simulink model "ACC_FFNN_trainbfg_30_30_30_Nor_Sat_Jan_24_RepFast"  (R2021a)
settings: Solver=FixedStepAuto  StartTime=0.0  StopTime=T  RelTol=1e-3
InitFcn:
  | seed = randi(10000);
StartFcn:
  | seed = randi(10000);
undefined symbols (not defined in the file): amax_ego, amin_ego, patch_sig, safe_patch_sig, sw, t_gap, Ts, v0_ego, v0_lead, v_set, x0_ego, x0_lead, x_gain, x_offset, y_gain, y_offset
libraries: neural x95, simulink x3
(part 1 of 5)
settings Model: Creator=The MathWorks, Inc.  LastModifiedBy=deyun
settings SolverCC: AlgebraicLoopSolver=TrustRegion
settings DataIOCC: ReturnWorkspaceOutputs=off
settings DebuggingCC: ArithmeticOperatorsInVariantConditions=warning
settings SFSimCC: SimUseLocalCustomCode=off  CustomCodeUndefinedFunction=UseInterfaceOnly
settings RTWCC: RTWUseLocalCustomCode=off
settings CodeAppCC: StateflowObjectComments=on
settings ConfigComp: CovBoundaryAbsTol=1.0e-5

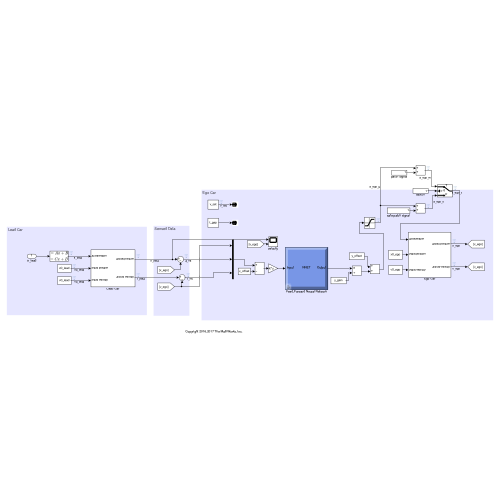
[thumbnail: Simulink's stored preview of the top-level diagram]
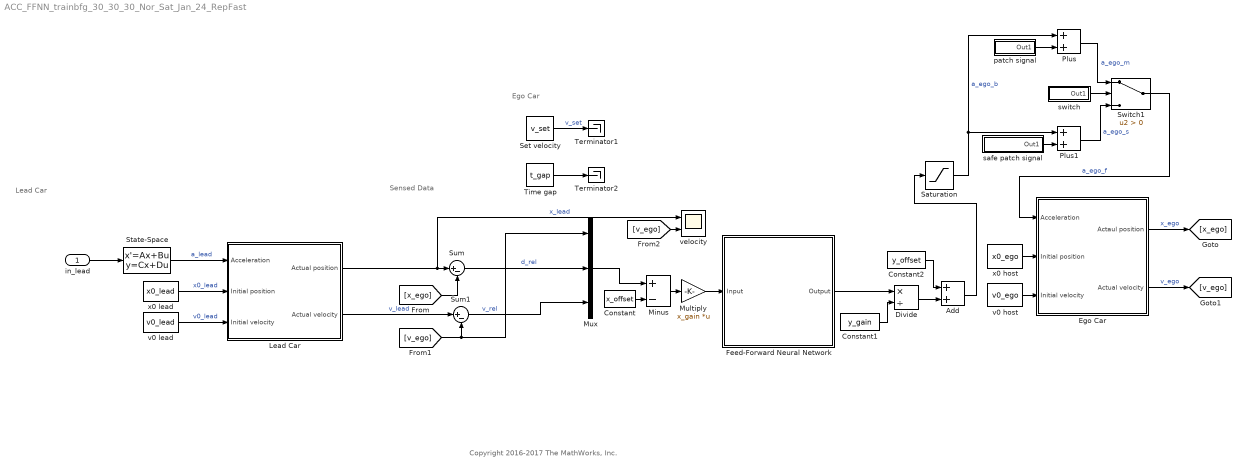
== system ACC_FFNN_trainbfg_30_30_30_Nor_Sat_Jan_24_RepFast ==
  note: Sensed Data
  note: Lead Car
  note: Ego Car
  note: Copyright 2016-2017 The MathWorks, Inc.
  in_lead : Inport
  Add : Sum
  Constant : Constant  Value=x_offset
  Constant1 : Constant  Value=y_gain
  Constant2 : Constant  Value=y_offset
  Divide : Product  Inputs=*/
  Ego Car : Subsystem
  Feed-Forward Neural Network : Subsystem
      mask help: Feed-Forward Neural Network
      mask Display: e = 0.06;c1 = [120 150 230]/255;c2 = ([120 150 230]+0)/383;c3 = ([120 150 230]+128)/383;patch([0 1 1 0],[0 0 1 1],c1);patch([0 1 1 1-e 1-e 0+e],[0 0 1 1-e 0+e 0+e],c2);patch([0 0 1 1-e 0+e 0+e],[0 1 1 1-e 1-e 0+e],c3);plot([0 1 1 0 0],[0 0 1 1 0]);fprintf('NNET');port_label('input',1,' Input');port_label('output',1,'Output ');
  Lead Car : Subsystem
  Minus : Sum  Inputs=+-
  Multiply : Gain  Gain=x_gain  Multiplication=Matrix(K*u)
  Mux : Mux  Inputs=3
  Plus : Sum
  Plus1 : Sum
  Saturation : Saturate  UpperLimit=amax_ego  LowerLimit=amin_ego
  Set velocity : Constant  Value=v_set  SampleTime=Ts
  State-Space : StateSpace  A=-10  B=10  D=0  InitialCondition=0
  Sum : Sum  Inputs=|+-
  Sum1 : Sum  Inputs=|+-
  Switch1 : Switch  Criteria=u2 > Threshold
  Terminator1 : Terminator
  Terminator2 : Terminator
  Time gap : Constant  Value=t_gap  SampleTime=Ts
  patch signal : Subsystem
  safe patch signal : Subsystem
  switch : Subsystem
  v0 host : Constant  Value=v0_ego  SampleTime=Ts
  v0 lead : Constant  Value=v0_lead  SampleTime=Ts
  velocity : Scope  NumInputPorts=2
  x0 host : Constant  Value=x0_ego  SampleTime=Ts
  x0 lead : Constant  Value=x0_lead  SampleTime=Ts
  wires:
  x0 lead/1 -> Lead Car/2(Initial position)  "x0_lead"
  v0 lead/1 -> Lead Car/3(Initial velocity)  "v0_lead"
  x0 host/1 -> Ego Car/2(Initial position)
  v0 host/1 -> Ego Car/3(Initial velocity)
  Feed-Forward Neural Network/1(Output) -> Divide/1
  Lead Car/1(Actual position) -> velocity/1, Sum/1  "x_lead"
  Sum1/1 -> Mux/3  "v_rel"
  State-Space/1 -> Lead Car/1(Acceleration)  "a_lead"
  Lead Car/2(Actual velocity) -> Sum1/1  "v_lead"
  in_lead/1 -> State-Space/1
  Mux/1 -> Minus/1
  Add/1 -> Saturation/1
  Multiply/1 -> Feed-Forward Neural Network/1(Input)
  Set velocity/1 -> Terminator1/1  "v_set"
  Time gap/1 -> Terminator2/1
  Constant/1 -> Minus/2
  Minus/1 -> Multiply/1
  Constant1/1 -> Divide/2
  Divide/1 -> Add/2
  Constant2/1 -> Add/1
  Ego Car/1(Actaul position) -> [x_ego]  "x_ego"
  [x_ego] -> Sum/2
  Ego Car/2(Actual velocity) -> [v_ego]  "v_ego"
  [v_ego] -> Mux/1, Sum1/2
  [v_ego] -> velocity/2
  Sum/1 -> Mux/2  "d_rel"
  Plus/1 -> Switch1/1  "a_ego_m"
  Plus1/1 -> Switch1/3  "a_ego_s"
  Switch1/1 -> Ego Car/1(Acceleration)  "a_ego_f"
  Saturation/1 -> Plus/1, Plus1/1  "a_ego_b"
  patch signal/1(Out1) -> Plus/2
  safe patch signal/1(Out1) -> Plus1/2
  switch/1(Out1) -> Switch1/2

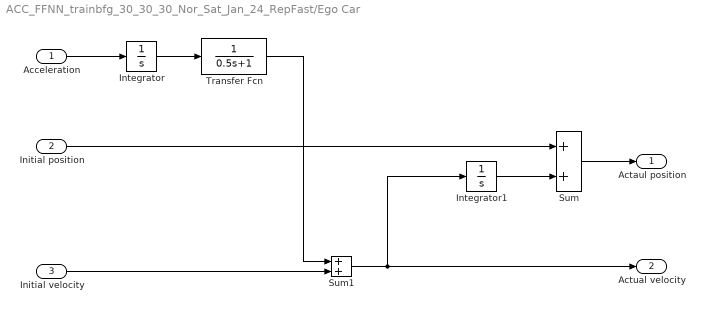
== system ACC_FFNN_trainbfg_30_30_30_Nor_Sat_Jan_24_RepFast/Ego Car ==
  Acceleration : Inport
  Initial position : Inport  Port=2
  Initial velocity : Inport  Port=3
  Integrator : Integrator
  Integrator1 : Integrator
  Sum : Sum
  Sum1 : Sum
  Transfer Fcn : TransferFcn  Denominator=[0.5 1]
  Actaul position : Outport  VectorParamsAs1DForOutWhenUnconnected=off
  Actual velocity : Outport  Port=2  VectorParamsAs1DForOutWhenUnconnected=off
  wires:
  Sum1/1 -> Integrator1/1, Actual velocity/1
  Initial velocity/1 -> Sum1/2
  Sum/1 -> Actaul position/1
  Transfer Fcn/1 -> Sum1/1
  Integrator/1 -> Transfer Fcn/1
  Acceleration/1 -> Integrator/1
  Initial position/1 -> Sum/1
  Integrator1/1 -> Sum/2

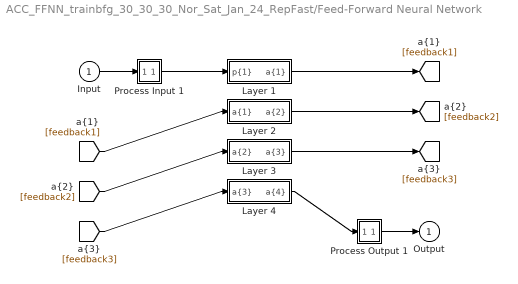
== system ACC_FFNN_trainbfg_30_30_30_Nor_Sat_Jan_24_RepFast/Feed-Forward Neural Network ==
  Input : Inport  PortDimensions=3
      mask Display: e = 0.06;c1 = [120 230 180]/255;c2 = ([120 230 180]+0)/(256+128);c3 = ([120 230 180]+128)/(256+128);patch([0 1 1 0],[0 0 1 1],c1);patch([0 1 1 1-e 1-e 0+e],[0 0 1 1-e 0+e 0+e],c2);patch([0 0 1 1-e 0+e 0+e],[0 1 1 1-e 1-e 0+e],c3);plot([0 1 1 0 0],[0 0 1 1 0]);
  Layer 1 : Subsystem
      mask Display: e = 0.06;c1 = [120 150 230]/255;c2 = ([120 150 230]+0)/383;c3 = ([120 150 230]+128)/383;patch([0 1 1 0],[0 0 1 1],c1);patch([0 1 1 1-e 1-e 0+e],[0 0 1 1-e 0+e 0+e],c2);patch([0 0 1 1-e 0+e 0+e],[0 1 1 1-e 1-e 0+e],c3);plot([0 1 1 0 0],[0 0 1 1 0]);
  Layer 2 : Subsystem
      mask Display: e = 0.06;c1 = [120 150 230]/255;c2 = ([120 150 230]+0)/383;c3 = ([120 150 230]+128)/383;patch([0 1 1 0],[0 0 1 1],c1);patch([0 1 1 1-e 1-e 0+e],[0 0 1 1-e 0+e 0+e],c2);patch([0 0 1 1-e 0+e 0+e],[0 1 1 1-e 1-e 0+e],c3);plot([0 1 1 0 0],[0 0 1 1 0]);
  Layer 3 : Subsystem
      mask Display: e = 0.06;c1 = [120 150 230]/255;c2 = ([120 150 230]+0)/383;c3 = ([120 150 230]+128)/383;patch([0 1 1 0],[0 0 1 1],c1);patch([0 1 1 1-e 1-e 0+e],[0 0 1 1-e 0+e 0+e],c2);patch([0 0 1 1-e 0+e 0+e],[0 1 1 1-e 1-e 0+e],c3);plot([0 1 1 0 0],[0 0 1 1 0]);
  Layer 4 : Subsystem
      mask Display: e = 0.06;c1 = [120 150 230]/255;c2 = ([120 150 230]+0)/383;c3 = ([120 150 230]+128)/383;patch([0 1 1 0],[0 0 1 1],c1);patch([0 1 1 1-e 1-e 0+e],[0 0 1 1-e 0+e 0+e],c2);patch([0 0 1 1-e 0+e 0+e],[0 1 1 1-e 1-e 0+e],c3);plot([0 1 1 0 0],[0 0 1 1 0]);
  Process Input 1 : Subsystem
      mask Display: e = 0.06;c1 = [120 150 230]/255;c2 = ([120 150 230]+0)/383;c3 = ([120 150 230]+128)/383;patch([0 1 1 0],[0 0 1 1],c1);patch([0 1 1 1-e 1-e 0+e],[0 0 1 1-e 0+e 0+e],c2);patch([0 0 1 1-e 0+e 0+e],[0 1 1 1-e 1-e 0+e],c3);plot([0 1 1 0 0],[0 0 1 1 0]);
  Process Output 1 : Subsystem
      mask Display: e = 0.06;c1 = [120 150 230]/255;c2 = ([120 150 230]+0)/383;c3 = ([120 150 230]+128)/383;patch([0 1 1 0],[0 0 1 1],c1);patch([0 1 1 1-e 1-e 0+e],[0 0 1 1-e 0+e 0+e],c2);patch([0 0 1 1-e 0+e 0+e],[0 1 1 1-e 1-e 0+e],c3);plot([0 1 1 0 0],[0 0 1 1 0]);
  Output : Outport  InitialOutput=0
      mask Display: e = 0.06;c1 = [120 230 180]/255;c2 = ([120 230 180]+0)/(256+128);c3 = ([120 230 180]+128)/(256+128);patch([0 1 1 0],[0 0 1 1],c1);patch([0 1 1 1-e 1-e 0+e],[0 0 1 1-e 0+e 0+e],c2);patch([0 0 1 1-e 0+e 0+e],[0 1 1 1-e 1-e 0+e],c3);plot([0 1 1 0 0],[0 0 1 1 0]);
  wires:
  Input/1 -> Process Input 1/1(x)
  Process Output 1/1(y) -> Output/1
  Process Input 1/1(p) -> Layer 1/1("p{1}")
  Layer 1/1("a{1}") -> [feedback1]
  [feedback1] -> Layer 2/1("a{1} ")
  Layer 2/1("a{2}") -> [feedback2]
  [feedback2] -> Layer 3/1("a{2} ")
  Layer 3/1("a{3}") -> [feedback3]
  [feedback3] -> Layer 4/1("a{3} ")
  Layer 4/1("a{4}") -> Process Output 1/1(a)

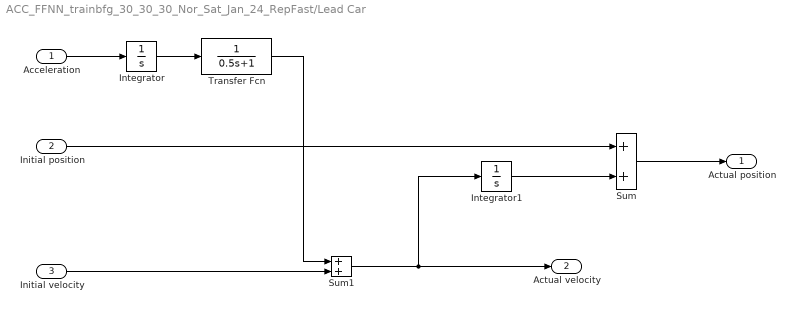
== system ACC_FFNN_trainbfg_30_30_30_Nor_Sat_Jan_24_RepFast/Lead Car ==
  Acceleration : Inport
  Initial position : Inport  Port=2
  Initial velocity : Inport  Port=3
  Integrator : Integrator
  Integrator1 : Integrator
  Sum : Sum
  Sum1 : Sum
  Transfer Fcn : TransferFcn  Denominator=[0.5 1]
  Actual position : Outport  VectorParamsAs1DForOutWhenUnconnected=off
  Actual velocity : Outport  Port=2  VectorParamsAs1DForOutWhenUnconnected=off
  wires:
  Transfer Fcn/1 -> Sum1/1
  Initial velocity/1 -> Sum1/2
  Sum/1 -> Actual position/1
  Integrator/1 -> Transfer Fcn/1
  Sum1/1 -> Integrator1/1, Actual velocity/1
  Acceleration/1 -> Integrator/1
  Initial position/1 -> Sum/1
  Integrator1/1 -> Sum/2

== system ACC_FFNN_trainbfg_30_30_30_Nor_Sat_Jan_24_RepFast/patch signal ==
  Sample index : simulink/Sources/Counter Limited  uplimit=numel(patch_sig)-1  tsamp=Ts
  Sample value : LookupNDDirect  NumberOfTableDimensions=1  Table=patch_sig  DiagnosticForOutOfRangeInput=None
  Out1 : Outport
  wires:
  Sample index/1 -> Sample value/1
  Sample value/1 -> Out1/1

== system ACC_FFNN_trainbfg_30_30_30_Nor_Sat_Jan_24_RepFast/safe patch signal ==
  Sample index : simulink/Sources/Counter Limited  uplimit=numel(safe_patch_sig)-1  tsamp=Ts
  Sample value : LookupNDDirect  NumberOfTableDimensions=1  Table=safe_patch_sig  DiagnosticForOutOfRangeInput=None
  Out1 : Outport
  wires:
  Sample index/1 -> Sample value/1
  Sample value/1 -> Out1/1

== system ACC_FFNN_trainbfg_30_30_30_Nor_Sat_Jan_24_RepFast/switch ==
  Sample index : simulink/Sources/Counter Limited  uplimit=numel(sw)-1  tsamp=Ts
  Sample value : LookupNDDirect  NumberOfTableDimensions=1  Table=sw  DiagnosticForOutOfRangeInput=None
  Out1 : Outport
  wires:
  Sample index/1 -> Sample value/1
  Sample value/1 -> Out1/1

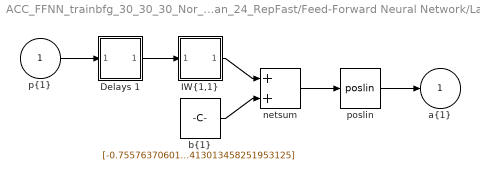
== system ACC_FFNN_trainbfg_30_30_30_Nor_Sat_Jan_24_RepFast/Feed-Forward Neural Network/Layer 1 ==
  "p{1}" : Inport  PortDimensions=3
      mask Display: e = 0.06;c1 = [120 230 180]/255;c2 = ([120 230 180]+0)/(256+128);c3 = ([120 230 180]+128)/(256+128);patch([0 1 1 0],[0 0 1 1],c1);patch([0 1 1 1-e 1-e 0+e],[0 0 1 1-e 0+e 0+e],c2);patch([0 0 1 1-e 0+e 0+e],[0 1 1 1-e 1-e 0+e],c3);plot([0 1 1 0 0],[0 0 1 1 0]);
  Delays 1 : Subsystem
      mask Display: e = 0.06;c1 = [120 150 230]/255;c2 = ([120 150 230]+0)/383;c3 = ([120 150 230]+128)/383;patch([0 1 1 0],[0 0 1 1],c1);patch([0 1 1 1-e 1-e 0+e],[0 0 1 1-e 0+e 0+e],c2);patch([0 0 1 1-e 0+e 0+e],[0 1 1 1-e 1-e 0+e],c3);plot([0 1 1 0 0],[0 0 1 1 0]);disp('0');
  "IW{1,1}" : Subsystem
      mask Display: e = 0.06;c1 = [120 150 230]/255;c2 = ([120 150 230]+0)/383;c3 = ([120 150 230]+128)/383;patch([0 1 1 0],[0 0 1 1],c1);patch([0 1 1 1-e 1-e 0+e],[0 0 1 1-e 0+e 0+e],c2);patch([0 0 1 1-e 0+e 0+e],[0 1 1 1-e 1-e 0+e],c3);plot([0 1 1 0 0],[0 0 1 1 0]);disp('W');
  "b{1}" : Constant  Value=[-0.75576370601788145364707816042937338352203369140625;0.2083910831518116790750383415797841735184192657470703125;-0.375365141914419719881834680563770234584808349609375;-0.9892272022507133666380241265869699418544769287109375;-0.0913594265985919473660459289021673612296581268310546875;-0.07369610707017504314109146434930153191089630126953125;-0.45364920227661276186381655861623585224151611328125;-0.3147913308418714972702900922740809619426727294921875;-0.5336188365404217481824389324174262583255767822265625;1.623775803722062871514708604081533849239349365234375;0.3355795759715054504823683600989170372486114501953125;1.1051526726069333950164264024351723492145538330078125;0.81244598487633268302232636415283195674419403076171875;-0.9907144071193039192024798467173241078853607177734375;-0.11998185237281365489447892969110398553311824798583984375;-0.6322641803625519418829981077578850090503692626953125;1.5229949158210016602055247858515940606594085693359375;-0.169937780238647473396440545911900699138641357421875;0.54861706405415378018375349711277522146701812744140625;-0.9371818138704508527325742761604487895965576171875;1.6474507840885854736967530698166228830814361572265625;0.21312299808273171830563796902424655854701995849609375;-0.02862398467868498830313228609156794846057891845703125;-0.775173406967106348730567333404906094074249267578125;0.5515881143870069447388004846288822591304779052734375;-0.2122678056651690070566473877988755702972412109375;0.94578193772742469302983181478339247405529022216796875;0.461704128067075669772378887500963173806667327880859375;1.1635521898512808380843353006639517843723297119140625;0.1472258131072077536050102253284421749413013458251953125]
      mask Display: e = 0.06;c1 = [120 150 230]/255;c2 = ([120 150 230]+0)/383;c3 = ([120 150 230]+128)/383;patch([0 1 1 0],[0 0 1 1],c1);patch([0 1 1 1-e 1-e 0+e],[0 0 1 1-e 0+e 0+e],c2);patch([0 0 1 1-e 0+e 0+e],[0 1 1 1-e 1-e 0+e],c3);plot([0 1 1 0 0],[0 0 1 1 0]);disp('b');
  netsum : Sum  Inputs=2  InputSameDT=on  SaturateOnIntegerOverflow=on  OutDataTypeStr=Inherit: Same as first input
      mask Display: e = 0.06;c1 = [120 150 230]/255;c2 = ([120 150 230]+0)/383;c3 = ([120 150 230]+128)/383;patch([0 1 1 0],[0 0 1 1],c1);patch([0 1 1 1-e 1-e 0+e],[0 0 1 1-e 0+e 0+e],c2);patch([0 0 1 1-e 0+e 0+e],[0 1 1 1-e 1-e 0+e],c3);plot([0 1 1 0 0],[0 0 1 1 0]);disp('+');
  poslin : neural/Transfer Functions/poslin
  "a{1}" : Outport  InitialOutput=[0;0;0;0;0;0;0;0;0;0;0;0;0;0;0;0;0;0;0;0;0;0;0;0;0;0;0;0;0;0]
      mask Display: e = 0.06;c1 = [120 230 180]/255;c2 = ([120 230 180]+0)/(256+128);c3 = ([120 230 180]+128)/(256+128);patch([0 1 1 0],[0 0 1 1],c1);patch([0 1 1 1-e 1-e 0+e],[0 0 1 1-e 0+e 0+e],c2);patch([0 0 1 1-e 0+e 0+e],[0 1 1 1-e 1-e 0+e],c3);plot([0 1 1 0 0],[0 0 1 1 0]);
  wires:
  "p{1}"/1 -> Delays 1/1("p{1}")
  Delays 1/1("pd{1,1}") -> "IW{1,1}"/1("pd{1,1}")
  "IW{1,1}"/1("iz{1,1}") -> netsum/1
  "b{1}"/1 -> netsum/2
  netsum/1 -> poslin/1
  poslin/1 -> "a{1}"/1

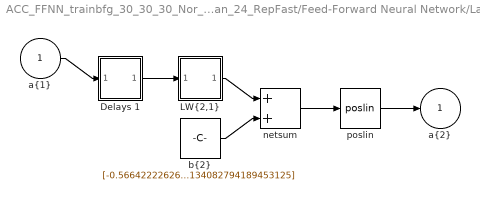
== system ACC_FFNN_trainbfg_30_30_30_Nor_Sat_Jan_24_RepFast/Feed-Forward Neural Network/Layer 2 ==
  "a{1} " : Inport  PortDimensions=30
      mask Display: e = 0.06;c1 = [120 230 180]/255;c2 = ([120 230 180]+0)/(256+128);c3 = ([120 230 180]+128)/(256+128);patch([0 1 1 0],[0 0 1 1],c1);patch([0 1 1 1-e 1-e 0+e],[0 0 1 1-e 0+e 0+e],c2);patch([0 0 1 1-e 0+e 0+e],[0 1 1 1-e 1-e 0+e],c3);plot([0 1 1 0 0],[0 0 1 1 0]);
  Delays 1 : Subsystem
      mask Display: e = 0.06;c1 = [120 150 230]/255;c2 = ([120 150 230]+0)/383;c3 = ([120 150 230]+128)/383;patch([0 1 1 0],[0 0 1 1],c1);patch([0 1 1 1-e 1-e 0+e],[0 0 1 1-e 0+e 0+e],c2);patch([0 0 1 1-e 0+e 0+e],[0 1 1 1-e 1-e 0+e],c3);plot([0 1 1 0 0],[0 0 1 1 0]);disp('0');
  "LW{2,1}" : Subsystem
      mask Display: e = 0.06;c1 = [120 150 230]/255;c2 = ([120 150 230]+0)/383;c3 = ([120 150 230]+128)/383;patch([0 1 1 0],[0 0 1 1],c1);patch([0 1 1 1-e 1-e 0+e],[0 0 1 1-e 0+e 0+e],c2);patch([0 0 1 1-e 0+e 0+e],[0 1 1 1-e 1-e 0+e],c3);plot([0 1 1 0 0],[0 0 1 1 0]);disp('W');
  "b{2}" : Constant  Value=[-0.5664222262670766117054199639824219048023223876953125;-0.21205392032648029410069057121290825307369232177734375;0.8902953437403631209434706761385314166545867919921875;-0.35341717925451254789237509612576104700565338134765625;1.817718697535364302808602587901987135410308837890625;0.0305090372892795162751422566316250595264136791229248046875;0.10985015507088920216904881499431212432682514190673828125;-0.80225146823424342557018462684936821460723876953125;-0.91799245781321492376747528396663255989551544189453125;-0.628537623354552987819943155045621097087860107421875;0.1343947896103030448244908257038332521915435791015625;-0.055194918880330623434105064006871543824672698974609375;0.343399503038541442645481538420426659286022186279296875;-0.4032848866040843471836296885157935321331024169921875;0.551385896889695192868430240196175873279571533203125;-0.5282221150190149483449886247399263083934783935546875;0.377796702150560548272295591232250444591045379638671875;-0.47239362807154716694668650234234519302845001220703125;0.33799719628211499777847848235978744924068450927734375;-0.0487780452192472235850573269999586045742034912109375;0.72237601794110550823546645915484987199306488037109375;0.954690941978406204526663714204914867877960205078125;-0.18570865551603177312500747575541026890277862548828125;-0.18708309364066533220238852663896977901458740234375;0.2024124955429655592364923677450860850512981414794921875;0.4283706057651504028882527563837356865406036376953125;0.8121838823116032113347273480030708014965057373046875;-0.528566935960145034556489918031729757785797119140625;-0.154096815674998943723750244316761381924152374267578125;0.6000992497267720882092589818057604134082794189453125]
      mask Display: e = 0.06;c1 = [120 150 230]/255;c2 = ([120 150 230]+0)/383;c3 = ([120 150 230]+128)/383;patch([0 1 1 0],[0 0 1 1],c1);patch([0 1 1 1-e 1-e 0+e],[0 0 1 1-e 0+e 0+e],c2);patch([0 0 1 1-e 0+e 0+e],[0 1 1 1-e 1-e 0+e],c3);plot([0 1 1 0 0],[0 0 1 1 0]);disp('b');
  netsum : Sum  Inputs=2  InputSameDT=on  SaturateOnIntegerOverflow=on  OutDataTypeStr=Inherit: Same as first input
      mask Display: e = 0.06;c1 = [120 150 230]/255;c2 = ([120 150 230]+0)/383;c3 = ([120 150 230]+128)/383;patch([0 1 1 0],[0 0 1 1],c1);patch([0 1 1 1-e 1-e 0+e],[0 0 1 1-e 0+e 0+e],c2);patch([0 0 1 1-e 0+e 0+e],[0 1 1 1-e 1-e 0+e],c3);plot([0 1 1 0 0],[0 0 1 1 0]);disp('+');
  poslin : neural/Transfer Functions/poslin
  "a{2}" : Outport  InitialOutput=[0;0;0;0;0;0;0;0;0;0;0;0;0;0;0;0;0;0;0;0;0;0;0;0;0;0;0;0;0;0]
      mask Display: e = 0.06;c1 = [120 230 180]/255;c2 = ([120 230 180]+0)/(256+128);c3 = ([120 230 180]+128)/(256+128);patch([0 1 1 0],[0 0 1 1],c1);patch([0 1 1 1-e 1-e 0+e],[0 0 1 1-e 0+e 0+e],c2);patch([0 0 1 1-e 0+e 0+e],[0 1 1 1-e 1-e 0+e],c3);plot([0 1 1 0 0],[0 0 1 1 0]);
  wires:
  "a{1} "/1 -> Delays 1/1("p{2}")
  Delays 1/1("pd{2,1}") -> "LW{2,1}"/1("ad{2,1}")
  "LW{2,1}"/1("lz{2,1}") -> netsum/1
  "b{2}"/1 -> netsum/2
  netsum/1 -> poslin/1
  poslin/1 -> "a{2}"/1

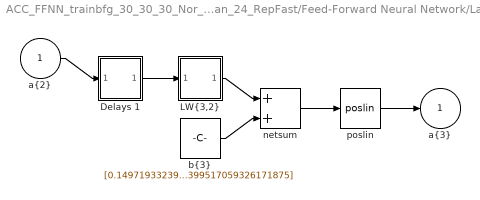
== system ACC_FFNN_trainbfg_30_30_30_Nor_Sat_Jan_24_RepFast/Feed-Forward Neural Network/Layer 3 ==
  "a{2} " : Inport  PortDimensions=30
      mask Display: e = 0.06;c1 = [120 230 180]/255;c2 = ([120 230 180]+0)/(256+128);c3 = ([120 230 180]+128)/(256+128);patch([0 1 1 0],[0 0 1 1],c1);patch([0 1 1 1-e 1-e 0+e],[0 0 1 1-e 0+e 0+e],c2);patch([0 0 1 1-e 0+e 0+e],[0 1 1 1-e 1-e 0+e],c3);plot([0 1 1 0 0],[0 0 1 1 0]);
  Delays 1 : Subsystem
      mask Display: e = 0.06;c1 = [120 150 230]/255;c2 = ([120 150 230]+0)/383;c3 = ([120 150 230]+128)/383;patch([0 1 1 0],[0 0 1 1],c1);patch([0 1 1 1-e 1-e 0+e],[0 0 1 1-e 0+e 0+e],c2);patch([0 0 1 1-e 0+e 0+e],[0 1 1 1-e 1-e 0+e],c3);plot([0 1 1 0 0],[0 0 1 1 0]);disp('0');
  "LW{3,2}" : Subsystem
      mask Display: e = 0.06;c1 = [120 150 230]/255;c2 = ([120 150 230]+0)/383;c3 = ([120 150 230]+128)/383;patch([0 1 1 0],[0 0 1 1],c1);patch([0 1 1 1-e 1-e 0+e],[0 0 1 1-e 0+e 0+e],c2);patch([0 0 1 1-e 0+e 0+e],[0 1 1 1-e 1-e 0+e],c3);plot([0 1 1 0 0],[0 0 1 1 0]);disp('W');
  "b{3}" : Constant  Value=[0.14971933239336099319416462094523012638092041015625;0.1417933436920632839228773036666098050773143768310546875;-0.06367538745269706035312395897562964819371700286865234375;-0.44516272996372208137216830436955206096172332763671875;-0.2218140399932438111552102100176853127777576446533203125;0.1863761903787369000884410752405528910458087921142578125;-0.96755766269959175840398302170797251164913177490234375;-0.897688716132796660218673423514701426029205322265625;0.96780661849546223418627732826280407607555389404296875;0.212261316933837207443502848036587238311767578125;-0.98552423327017157905771682635531760752201080322265625;0.09653335078981058192670872131202486343681812286376953125;-0.2297805231487659305411597188140149228274822235107421875;0.022037172189857963389147954558211495168507099151611328125;-0.6562981059863186583669403262319974601268768310546875;0.0281456454940819424115350244619548902846872806549072265625;-0.13531390979653690198603044336778111755847930908203125;-0.392353844554378827780283245374448597431182861328125;-0.5461924787583296581061631513875909149646759033203125;-0.72148274854000504774376167915761470794677734375;-0.51434969025329502212429133578552864491939544677734375;-0.54014674630848824588014167602523230016231536865234375;0.498809806279932654859976537409238517284393310546875;0.61873481372022620661255132290534675121307373046875;0.292993921966925141564530576943070627748966217041015625;-0.46701088858658212910057727640378288924694061279296875;-0.321428784817516799421355244703590869903564453125;0.66359237271291515725124554592184722423553466796875;-0.59181063371320075106041258550249040126800537109375;0.5064617222498568605004720666329376399517059326171875]
      mask Display: e = 0.06;c1 = [120 150 230]/255;c2 = ([120 150 230]+0)/383;c3 = ([120 150 230]+128)/383;patch([0 1 1 0],[0 0 1 1],c1);patch([0 1 1 1-e 1-e 0+e],[0 0 1 1-e 0+e 0+e],c2);patch([0 0 1 1-e 0+e 0+e],[0 1 1 1-e 1-e 0+e],c3);plot([0 1 1 0 0],[0 0 1 1 0]);disp('b');
  netsum : Sum  Inputs=2  InputSameDT=on  SaturateOnIntegerOverflow=on  OutDataTypeStr=Inherit: Same as first input
      mask Display: e = 0.06;c1 = [120 150 230]/255;c2 = ([120 150 230]+0)/383;c3 = ([120 150 230]+128)/383;patch([0 1 1 0],[0 0 1 1],c1);patch([0 1 1 1-e 1-e 0+e],[0 0 1 1-e 0+e 0+e],c2);patch([0 0 1 1-e 0+e 0+e],[0 1 1 1-e 1-e 0+e],c3);plot([0 1 1 0 0],[0 0 1 1 0]);disp('+');
  poslin : neural/Transfer Functions/poslin
  "a{3}" : Outport  InitialOutput=[0;0;0;0;0;0;0;0;0;0;0;0;0;0;0;0;0;0;0;0;0;0;0;0;0;0;0;0;0;0]
      mask Display: e = 0.06;c1 = [120 230 180]/255;c2 = ([120 230 180]+0)/(256+128);c3 = ([120 230 180]+128)/(256+128);patch([0 1 1 0],[0 0 1 1],c1);patch([0 1 1 1-e 1-e 0+e],[0 0 1 1-e 0+e 0+e],c2);patch([0 0 1 1-e 0+e 0+e],[0 1 1 1-e 1-e 0+e],c3);plot([0 1 1 0 0],[0 0 1 1 0]);
  wires:
  "a{2} "/1 -> Delays 1/1("p{3}")
  Delays 1/1("pd{3,2}") -> "LW{3,2}"/1("ad{3,2}")
  "LW{3,2}"/1("lz{3,2}") -> netsum/1
  "b{3}"/1 -> netsum/2
  netsum/1 -> poslin/1
  poslin/1 -> "a{3}"/1

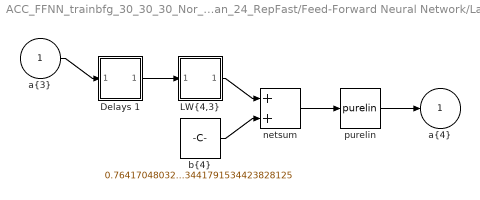
== system ACC_FFNN_trainbfg_30_30_30_Nor_Sat_Jan_24_RepFast/Feed-Forward Neural Network/Layer 4 ==
  "a{3} " : Inport  PortDimensions=30
      mask Display: e = 0.06;c1 = [120 230 180]/255;c2 = ([120 230 180]+0)/(256+128);c3 = ([120 230 180]+128)/(256+128);patch([0 1 1 0],[0 0 1 1],c1);patch([0 1 1 1-e 1-e 0+e],[0 0 1 1-e 0+e 0+e],c2);patch([0 0 1 1-e 0+e 0+e],[0 1 1 1-e 1-e 0+e],c3);plot([0 1 1 0 0],[0 0 1 1 0]);
  Delays 1 : Subsystem
      mask Display: e = 0.06;c1 = [120 150 230]/255;c2 = ([120 150 230]+0)/383;c3 = ([120 150 230]+128)/383;patch([0 1 1 0],[0 0 1 1],c1);patch([0 1 1 1-e 1-e 0+e],[0 0 1 1-e 0+e 0+e],c2);patch([0 0 1 1-e 0+e 0+e],[0 1 1 1-e 1-e 0+e],c3);plot([0 1 1 0 0],[0 0 1 1 0]);disp('0');
  "LW{4,3}" : Subsystem
      mask Display: e = 0.06;c1 = [120 150 230]/255;c2 = ([120 150 230]+0)/383;c3 = ([120 150 230]+128)/383;patch([0 1 1 0],[0 0 1 1],c1);patch([0 1 1 1-e 1-e 0+e],[0 0 1 1-e 0+e 0+e],c2);patch([0 0 1 1-e 0+e 0+e],[0 1 1 1-e 1-e 0+e],c3);plot([0 1 1 0 0],[0 0 1 1 0]);disp('W');
  "b{4}" : Constant  Value=0.7641704803230979781147880203207023441791534423828125
      mask Display: e = 0.06;c1 = [120 150 230]/255;c2 = ([120 150 230]+0)/383;c3 = ([120 150 230]+128)/383;patch([0 1 1 0],[0 0 1 1],c1);patch([0 1 1 1-e 1-e 0+e],[0 0 1 1-e 0+e 0+e],c2);patch([0 0 1 1-e 0+e 0+e],[0 1 1 1-e 1-e 0+e],c3);plot([0 1 1 0 0],[0 0 1 1 0]);disp('b');
  netsum : Sum  Inputs=2  InputSameDT=on  SaturateOnIntegerOverflow=on  OutDataTypeStr=Inherit: Same as first input
      mask Display: e = 0.06;c1 = [120 150 230]/255;c2 = ([120 150 230]+0)/383;c3 = ([120 150 230]+128)/383;patch([0 1 1 0],[0 0 1 1],c1);patch([0 1 1 1-e 1-e 0+e],[0 0 1 1-e 0+e 0+e],c2);patch([0 0 1 1-e 0+e 0+e],[0 1 1 1-e 1-e 0+e],c3);plot([0 1 1 0 0],[0 0 1 1 0]);disp('+');
  purelin : neural/Transfer Functions/purelin
  "a{4}" : Outport  InitialOutput=0
      mask Display: e = 0.06;c1 = [120 230 180]/255;c2 = ([120 230 180]+0)/(256+128);c3 = ([120 230 180]+128)/(256+128);patch([0 1 1 0],[0 0 1 1],c1);patch([0 1 1 1-e 1-e 0+e],[0 0 1 1-e 0+e 0+e],c2);patch([0 0 1 1-e 0+e 0+e],[0 1 1 1-e 1-e 0+e],c3);plot([0 1 1 0 0],[0 0 1 1 0]);
  wires:
  "a{3} "/1 -> Delays 1/1("p{4}")
  Delays 1/1("pd{4,3}") -> "LW{4,3}"/1("ad{4,3}")
  "LW{4,3}"/1("lz{4,3}") -> netsum/1
  "b{4}"/1 -> netsum/2
  netsum/1 -> purelin/1
  purelin/1 -> "a{4}"/1

== system ACC_FFNN_trainbfg_30_30_30_Nor_Sat_Jan_24_RepFast/Feed-Forward Neural Network/Process Input 1 ==
  x : Inport  PortDimensions=3
      mask Display: e = 0.06;c1 = [120 230 180]/255;c2 = ([120 230 180]+0)/(256+128);c3 = ([120 230 180]+128)/(256+128);patch([0 1 1 0],[0 0 1 1],c1);patch([0 1 1 1-e 1-e 0+e],[0 0 1 1-e 0+e 0+e],c2);patch([0 0 1 1-e 0+e 0+e],[0 1 1 1-e 1-e 0+e],c3);plot([0 1 1 0 0],[0 0 1 1 0]);
  p : Outport  PortDimensions=3
      mask Display: e = 0.06;c1 = [120 230 180]/255;c2 = ([120 230 180]+0)/(256+128);c3 = ([120 230 180]+128)/(256+128);patch([0 1 1 0],[0 0 1 1],c1);patch([0 1 1 1-e 1-e 0+e],[0 0 1 1-e 0+e 0+e],c2);patch([0 0 1 1-e 0+e 0+e],[0 1 1 1-e 1-e 0+e],c3);plot([0 1 1 0 0],[0 0 1 1 0]);
  wires:
  x/1 -> p/1

== system ACC_FFNN_trainbfg_30_30_30_Nor_Sat_Jan_24_RepFast/Feed-Forward Neural Network/Process Output 1 ==
  a : Inport  PortDimensions=1
      mask Display: e = 0.06;c1 = [120 230 180]/255;c2 = ([120 230 180]+0)/(256+128);c3 = ([120 230 180]+128)/(256+128);patch([0 1 1 0],[0 0 1 1],c1);patch([0 1 1 1-e 1-e 0+e],[0 0 1 1-e 0+e 0+e],c2);patch([0 0 1 1-e 0+e 0+e],[0 1 1 1-e 1-e 0+e],c3);plot([0 1 1 0 0],[0 0 1 1 0]);
  y : Outport  PortDimensions=1
      mask Display: e = 0.06;c1 = [120 230 180]/255;c2 = ([120 230 180]+0)/(256+128);c3 = ([120 230 180]+128)/(256+128);patch([0 1 1 0],[0 0 1 1],c1);patch([0 1 1 1-e 1-e 0+e],[0 0 1 1-e 0+e 0+e],c2);patch([0 0 1 1-e 0+e 0+e],[0 1 1 1-e 1-e 0+e],c3);plot([0 1 1 0 0],[0 0 1 1 0]);
  wires:
  a/1 -> y/1

== system ACC_FFNN_trainbfg_30_30_30_Nor_Sat_Jan_24_RepFast/Feed-Forward Neural Network/Layer 1/Delays 1 ==
  "p{1}" : Inport  PortDimensions=3
      mask Display: e = 0.06;c1 = [120 230 180]/255;c2 = ([120 230 180]+0)/(256+128);c3 = ([120 230 180]+128)/(256+128);patch([0 1 1 0],[0 0 1 1],c1);patch([0 1 1 1-e 1-e 0+e],[0 0 1 1-e 0+e 0+e],c2);patch([0 0 1 1-e 0+e 0+e],[0 1 1 1-e 1-e 0+e],c3);plot([0 1 1 0 0],[0 0 1 1 0]);
  mux : Mux  Inputs=1
      mask Display: e = 0.06;c1 = [120 150 230]/255;c2 = ([120 150 230]+0)/383;c3 = ([120 150 230]+128)/383;patch([0 1 1 0],[0 0 1 1],c1);patch([0 1 1 1-e 1-e 0+e],[0 0 1 1-e 0+e 0+e],c2);patch([0 0 1 1-e 0+e 0+e],[0 1 1 1-e 1-e 0+e],c3);plot([0 1 1 0 0],[0 0 1 1 0]);disp('Mux')
  "pd{1,1}" : Outport
      mask Display: e = 0.06;c1 = [120 230 180]/255;c2 = ([120 230 180]+0)/(256+128);c3 = ([120 230 180]+128)/(256+128);patch([0 1 1 0],[0 0 1 1],c1);patch([0 1 1 1-e 1-e 0+e],[0 0 1 1-e 0+e 0+e],c2);patch([0 0 1 1-e 0+e 0+e],[0 1 1 1-e 1-e 0+e],c3);plot([0 1 1 0 0],[0 0 1 1 0]);
  wires:
  "p{1}"/1 -> mux/1
  mux/1 -> "pd{1,1}"/1

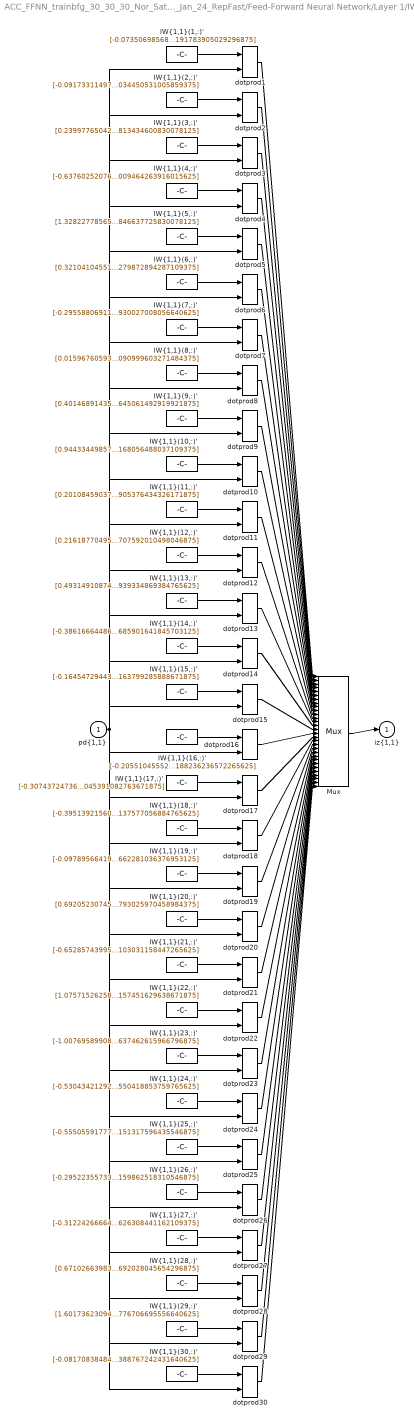
== system ACC_FFNN_trainbfg_30_30_30_Nor_Sat_Jan_24_RepFast/Feed-Forward Neural Network/Layer 1/IW{1,1} ==
  "pd{1,1}" : Inport  PortDimensions=3
      mask Display: e = 0.06;c1 = [120 230 180]/255;c2 = ([120 230 180]+0)/(256+128);c3 = ([120 230 180]+128)/(256+128);patch([0 1 1 0],[0 0 1 1],c1);patch([0 1 1 1-e 1-e 0+e],[0 0 1 1-e 0+e 0+e],c2);patch([0 0 1 1-e 0+e 0+e],[0 1 1 1-e 1-e 0+e],c3);plot([0 1 1 0 0],[0 0 1 1 0]);
  "IW{1,1}(1,:)'" : Constant  Value=[-0.0735069856879080330003262133686803281307220458984375;0.572746574072698688695481905597262084484100341796875;-0.468568101961270411237592270481400191783905029296875]
      mask Display: e = 0.06;c1 = [120 150 230]/255;c2 = ([120 150 230]+0)/383;c3 = ([120 150 230]+128)/383;patch([0 1 1 0],[0 0 1 1],c1);patch([0 1 1 1-e 1-e 0+e],[0 0 1 1-e 0+e 0+e],c2);patch([0 0 1 1-e 0+e 0+e],[0 1 1 1-e 1-e 0+e],c3);plot([0 1 1 0 0],[0 0 1 1 0]);disp('Weights');
  "IW{1,1}(10,:)'" : Constant  Value=[0.94433449857315299169613354024477303028106689453125;-2.023137587114056668013972739572636783123016357421875;0.62150667384027646900079844272113405168056488037109375]
      mask Display: e = 0.06;c1 = [120 150 230]/255;c2 = ([120 150 230]+0)/383;c3 = ([120 150 230]+128)/383;patch([0 1 1 0],[0 0 1 1],c1);patch([0 1 1 1-e 1-e 0+e],[0 0 1 1-e 0+e 0+e],c2);patch([0 0 1 1-e 0+e 0+e],[0 1 1 1-e 1-e 0+e],c3);plot([0 1 1 0 0],[0 0 1 1 0]);disp('Weights');
  "IW{1,1}(11,:)'" : Constant  Value=[0.201084590373814708907929116321611218154430389404296875;1.6547413112236724064274540069163776934146881103515625;0.81270947029375306680520907320897094905376434326171875]
      mask Display: e = 0.06;c1 = [120 150 230]/255;c2 = ([120 150 230]+0)/383;c3 = ([120 150 230]+128)/383;patch([0 1 1 0],[0 0 1 1],c1);patch([0 1 1 1-e 1-e 0+e],[0 0 1 1-e 0+e 0+e],c2);patch([0 0 1 1-e 0+e 0+e],[0 1 1 1-e 1-e 0+e],c3);plot([0 1 1 0 0],[0 0 1 1 0]);disp('Weights');
  "IW{1,1}(12,:)'" : Constant  Value=[0.2161877049575451348317756128381006419658660888671875;-0.61841255723046473224968622162123210728168487548828125;0.928308580390744708665806683711707592010498046875]
      mask Display: e = 0.06;c1 = [120 150 230]/255;c2 = ([120 150 230]+0)/383;c3 = ([120 150 230]+128)/383;patch([0 1 1 0],[0 0 1 1],c1);patch([0 1 1 1-e 1-e 0+e],[0 0 1 1-e 0+e 0+e],c2);patch([0 0 1 1-e 0+e 0+e],[0 1 1 1-e 1-e 0+e],c3);plot([0 1 1 0 0],[0 0 1 1 0]);disp('Weights');
  "IW{1,1}(13,:)'" : Constant  Value=[0.493149108744405484383577231710660271346569061279296875;-0.58041686117544755152408697540522553026676177978515625;0.289037279137445202170653146822587586939334869384765625]
      mask Display: e = 0.06;c1 = [120 150 230]/255;c2 = ([120 150 230]+0)/383;c3 = ([120 150 230]+128)/383;patch([0 1 1 0],[0 0 1 1],c1);patch([0 1 1 1-e 1-e 0+e],[0 0 1 1-e 0+e 0+e],c2);patch([0 0 1 1-e 0+e 0+e],[0 1 1 1-e 1-e 0+e],c3);plot([0 1 1 0 0],[0 0 1 1 0]);disp('Weights');
  "IW{1,1}(14,:)'" : Constant  Value=[-0.386166644862619257150271323553170077502727508544921875;0.442477595750223107184950777082121931016445159912109375;-0.46023184841021358426615961434436030685901641845703125]
      mask Display: e = 0.06;c1 = [120 150 230]/255;c2 = ([120 150 230]+0)/383;c3 = ([120 150 230]+128)/383;patch([0 1 1 0],[0 0 1 1],c1);patch([0 1 1 1-e 1-e 0+e],[0 0 1 1-e 0+e 0+e],c2);patch([0 0 1 1-e 0+e 0+e],[0 1 1 1-e 1-e 0+e],c3);plot([0 1 1 0 0],[0 0 1 1 0]);disp('Weights');
  "IW{1,1}(15,:)'" : Constant  Value=[-0.1645472944382107283178839907122892327606678009033203125;3.17897330010412826339916136930696666240692138671875;0.3414517110865318283430269730160944163799285888671875]
      mask Display: e = 0.06;c1 = [120 150 230]/255;c2 = ([120 150 230]+0)/383;c3 = ([120 150 230]+128)/383;patch([0 1 1 0],[0 0 1 1],c1);patch([0 1 1 1-e 1-e 0+e],[0 0 1 1-e 0+e 0+e],c2);patch([0 0 1 1-e 0+e 0+e],[0 1 1 1-e 1-e 0+e],c3);plot([0 1 1 0 0],[0 0 1 1 0]);disp('Weights');
  "IW{1,1}(16,:)'" : Constant  Value=[-0.205510455529933633300743167637847363948822021484375;0.9463349145633006553879340572166256606578826904296875;-0.546104741471600707569677979336120188236236572265625]
      mask Display: e = 0.06;c1 = [120 150 230]/255;c2 = ([120 150 230]+0)/383;c3 = ([120 150 230]+128)/383;patch([0 1 1 0],[0 0 1 1],c1);patch([0 1 1 1-e 1-e 0+e],[0 0 1 1-e 0+e 0+e],c2);patch([0 0 1 1-e 0+e 0+e],[0 1 1 1-e 1-e 0+e],c3);plot([0 1 1 0 0],[0 0 1 1 0]);disp('Weights');
  "IW{1,1}(17,:)'" : Constant  Value=[-0.30743724736218214221850075773545540869235992431640625;-1.5580123540270383042383173233247362077236175537109375;0.11148648289516631393336609789912472479045391082763671875]
      mask Display: e = 0.06;c1 = [120 150 230]/255;c2 = ([120 150 230]+0)/383;c3 = ([120 150 230]+128)/383;patch([0 1 1 0],[0 0 1 1],c1);patch([0 1 1 1-e 1-e 0+e],[0 0 1 1-e 0+e 0+e],c2);patch([0 0 1 1-e 0+e 0+e],[0 1 1 1-e 1-e 0+e],c3);plot([0 1 1 0 0],[0 0 1 1 0]);disp('Weights');
  "IW{1,1}(18,:)'" : Constant  Value=[-0.3951392156055018034521708614192903041839599609375;-0.234075053012488876191810049931518733501434326171875;0.4829374839064561886203819085494615137577056884765625]
      mask Display: e = 0.06;c1 = [120 150 230]/255;c2 = ([120 150 230]+0)/383;c3 = ([120 150 230]+128)/383;patch([0 1 1 0],[0 0 1 1],c1);patch([0 1 1 1-e 1-e 0+e],[0 0 1 1-e 0+e 0+e],c2);patch([0 0 1 1-e 0+e 0+e],[0 1 1 1-e 1-e 0+e],c3);plot([0 1 1 0 0],[0 0 1 1 0]);disp('Weights');
  "IW{1,1}(19,:)'" : Constant  Value=[-0.09789566419941275743354935912066139280796051025390625;2.544710393957738236991872327052988111972808837890625;0.333012836046979732174122545984573662281036376953125]
      mask Display: e = 0.06;c1 = [120 150 230]/255;c2 = ([120 150 230]+0)/383;c3 = ([120 150 230]+128)/383;patch([0 1 1 0],[0 0 1 1],c1);patch([0 1 1 1-e 1-e 0+e],[0 0 1 1-e 0+e 0+e],c2);patch([0 0 1 1-e 0+e 0+e],[0 1 1 1-e 1-e 0+e],c3);plot([0 1 1 0 0],[0 0 1 1 0]);disp('Weights');
  "IW{1,1}(2,:)'" : Constant  Value=[-0.09173311497974841188796091273616184480488300323486328125;-0.1317797854408500335399168079675291664898395538330078125;0.6627215975901135092129834447405301034450531005859375]
      mask Display: e = 0.06;c1 = [120 150 230]/255;c2 = ([120 150 230]+0)/383;c3 = ([120 150 230]+128)/383;patch([0 1 1 0],[0 0 1 1],c1);patch([0 1 1 1-e 1-e 0+e],[0 0 1 1-e 0+e 0+e],c2);patch([0 0 1 1-e 0+e 0+e],[0 1 1 1-e 1-e 0+e],c3);plot([0 1 1 0 0],[0 0 1 1 0]);disp('Weights');
  "IW{1,1}(20,:)'" : Constant  Value=[0.69205230745780621504081864259205758571624755859375;-0.5251550585759228173543533557676710188388824462890625;-0.2848081402893229974182531805126927793025970458984375]
      mask Display: e = 0.06;c1 = [120 150 230]/255;c2 = ([120 150 230]+0)/383;c3 = ([120 150 230]+128)/383;patch([0 1 1 0],[0 0 1 1],c1);patch([0 1 1 1-e 1-e 0+e],[0 0 1 1-e 0+e 0+e],c2);patch([0 0 1 1-e 0+e 0+e],[0 1 1 1-e 1-e 0+e],c3);plot([0 1 1 0 0],[0 0 1 1 0]);disp('Weights');
  "IW{1,1}(21,:)'" : Constant  Value=[-0.65285743995412348628093468505539931356906890869140625;-1.2173424004765134309735685747000388801097869873046875;0.68805145669451894807622238658950664103031158447265625]
      mask Display: e = 0.06;c1 = [120 150 230]/255;c2 = ([120 150 230]+0)/383;c3 = ([120 150 230]+128)/383;patch([0 1 1 0],[0 0 1 1],c1);patch([0 1 1 1-e 1-e 0+e],[0 0 1 1-e 0+e 0+e],c2);patch([0 0 1 1-e 0+e 0+e],[0 1 1 1-e 1-e 0+e],c3);plot([0 1 1 0 0],[0 0 1 1 0]);disp('Weights');
  "IW{1,1}(22,:)'" : Constant  Value=[1.075715262581673048458696939633227884769439697265625;2.846796183729652707228297003894113004207611083984375;0.74071874836254181229122650620411150157451629638671875]
      mask Display: e = 0.06;c1 = [120 150 230]/255;c2 = ([120 150 230]+0)/383;c3 = ([120 150 230]+128)/383;patch([0 1 1 0],[0 0 1 1],c1);patch([0 1 1 1-e 1-e 0+e],[0 0 1 1-e 0+e 0+e],c2);patch([0 0 1 1-e 0+e 0+e],[0 1 1 1-e 1-e 0+e],c3);plot([0 1 1 0 0],[0 0 1 1 0]);disp('Weights');
  "IW{1,1}(23,:)'" : Constant  Value=[-1.0076958990811386573938079891377128660678863525390625;0.9052568951862955959342116329935379326343536376953125;-0.7290251114562085188453011141973547637462615966796875]
      mask Display: e = 0.06;c1 = [120 150 230]/255;c2 = ([120 150 230]+0)/383;c3 = ([120 150 230]+128)/383;patch([0 1 1 0],[0 0 1 1],c1);patch([0 1 1 1-e 1-e 0+e],[0 0 1 1-e 0+e 0+e],c2);patch([0 0 1 1-e 0+e 0+e],[0 1 1 1-e 1-e 0+e],c3);plot([0 1 1 0 0],[0 0 1 1 0]);disp('Weights');
  "IW{1,1}(24,:)'" : Constant  Value=[-0.53043421292017922663575291153392754495143890380859375;-0.0285098552808798026692027605122348177246749401092529296875;0.786992736121922664693784099654294550418853759765625]
      mask Display: e = 0.06;c1 = [120 150 230]/255;c2 = ([120 150 230]+0)/383;c3 = ([120 150 230]+128)/383;patch([0 1 1 0],[0 0 1 1],c1);patch([0 1 1 1-e 1-e 0+e],[0 0 1 1-e 0+e 0+e],c2);patch([0 0 1 1-e 0+e 0+e],[0 1 1 1-e 1-e 0+e],c3);plot([0 1 1 0 0],[0 0 1 1 0]);disp('Weights');
  "IW{1,1}(25,:)'" : Constant  Value=[-0.55505591777922191898397841214318759739398956298828125;0.69988849495154659141604724936769343912601470947265625;-0.027605746880141383836626545189574244432151317596435546875]
      mask Display: e = 0.06;c1 = [120 150 230]/255;c2 = ([120 150 230]+0)/383;c3 = ([120 150 230]+128)/383;patch([0 1 1 0],[0 0 1 1],c1);patch([0 1 1 1-e 1-e 0+e],[0 0 1 1-e 0+e 0+e],c2);patch([0 0 1 1-e 0+e 0+e],[0 1 1 1-e 1-e 0+e],c3);plot([0 1 1 0 0],[0 0 1 1 0]);disp('Weights');
  "IW{1,1}(26,:)'" : Constant  Value=[-0.295223557338710751452026670449413359165191650390625;-0.0293963635355940500204496856895275413990020751953125;-0.2649257518324457105762803621473722159862518310546875]
      mask Display: e = 0.06;c1 = [120 150 230]/255;c2 = ([120 150 230]+0)/383;c3 = ([120 150 230]+128)/383;patch([0 1 1 0],[0 0 1 1],c1);patch([0 1 1 1-e 1-e 0+e],[0 0 1 1-e 0+e 0+e],c2);patch([0 0 1 1-e 0+e 0+e],[0 1 1 1-e 1-e 0+e],c3);plot([0 1 1 0 0],[0 0 1 1 0]);disp('Weights');
  "IW{1,1}(27,:)'" : Constant  Value=[-0.31224266664768929313567014105501584708690643310546875;0.9687520568497394179985349182970821857452392578125;0.89768516641125639665688140667043626308441162109375]
      mask Display: e = 0.06;c1 = [120 150 230]/255;c2 = ([120 150 230]+0)/383;c3 = ([120 150 230]+128)/383;patch([0 1 1 0],[0 0 1 1],c1);patch([0 1 1 1-e 1-e 0+e],[0 0 1 1-e 0+e 0+e],c2);patch([0 0 1 1-e 0+e 0+e],[0 1 1 1-e 1-e 0+e],c3);plot([0 1 1 0 0],[0 0 1 1 0]);disp('Weights');
  "IW{1,1}(28,:)'" : Constant  Value=[0.6710266398332940251947320575709454715251922607421875;0.74621757732697291398693550945608876645565032958984375;-0.587465278623997999574157802271656692028045654296875]
      mask Display: e = 0.06;c1 = [120 150 230]/255;c2 = ([120 150 230]+0)/383;c3 = ([120 150 230]+128)/383;patch([0 1 1 0],[0 0 1 1],c1);patch([0 1 1 1-e 1-e 0+e],[0 0 1 1-e 0+e 0+e],c2);patch([0 0 1 1-e 0+e 0+e],[0 1 1 1-e 1-e 0+e],c3);plot([0 1 1 0 0],[0 0 1 1 0]);disp('Weights');
  "IW{1,1}(29,:)'" : Constant  Value=[1.601736230947659489487477912916801869869232177734375;0.06740718394308080341215116959574515931308269500732421875;0.26242192674588837864035895108827389776706695556640625]
      mask Display: e = 0.06;c1 = [120 150 230]/255;c2 = ([120 150 230]+0)/383;c3 = ([120 150 230]+128)/383;patch([0 1 1 0],[0 0 1 1],c1);patch([0 1 1 1-e 1-e 0+e],[0 0 1 1-e 0+e 0+e],c2);patch([0 0 1 1-e 0+e 0+e],[0 1 1 1-e 1-e 0+e],c3);plot([0 1 1 0 0],[0 0 1 1 0]);disp('Weights');
  "IW{1,1}(3,:)'" : Constant  Value=[0.2399776504216930561597109772264957427978515625;0.2144585366630098466345089036622084677219390869140625;-0.2678446745286315877621063918923027813434600830078125]
      mask Display: e = 0.06;c1 = [120 150 230]/255;c2 = ([120 150 230]+0)/383;c3 = ([120 150 230]+128)/383;patch([0 1 1 0],[0 0 1 1],c1);patch([0 1 1 1-e 1-e 0+e],[0 0 1 1-e 0+e 0+e],c2);patch([0 0 1 1-e 0+e 0+e],[0 1 1 1-e 1-e 0+e],c3);plot([0 1 1 0 0],[0 0 1 1 0]);disp('Weights');
  "IW{1,1}(30,:)'" : Constant  Value=[-0.0817083848440221249820325510881957598030567169189453125;0.267809671869804810651061188764288090169429779052734375;0.246791544914894134254979007891961373388767242431640625]
      mask Display: e = 0.06;c1 = [120 150 230]/255;c2 = ([120 150 230]+0)/383;c3 = ([120 150 230]+128)/383;patch([0 1 1 0],[0 0 1 1],c1);patch([0 1 1 1-e 1-e 0+e],[0 0 1 1-e 0+e 0+e],c2);patch([0 0 1 1-e 0+e 0+e],[0 1 1 1-e 1-e 0+e],c3);plot([0 1 1 0 0],[0 0 1 1 0]);disp('Weights');
  "IW{1,1}(4,:)'" : Constant  Value=[-0.63760252076230294893122163557563908398151397705078125;0.233685575931445288500043488966184668242931365966796875;0.5211168660847447231532214573235251009464263916015625]
      mask Display: e = 0.06;c1 = [120 150 230]/255;c2 = ([120 150 230]+0)/383;c3 = ([120 150 230]+128)/383;patch([0 1 1 0],[0 0 1 1],c1);patch([0 1 1 1-e 1-e 0+e],[0 0 1 1-e 0+e 0+e],c2);patch([0 0 1 1-e 0+e 0+e],[0 1 1 1-e 1-e 0+e],c3);plot([0 1 1 0 0],[0 0 1 1 0]);disp('Weights');
  "IW{1,1}(5,:)'" : Constant  Value=[1.3282277856555573247732127128983847796916961669921875;0.315552112314307187102002671963418833911418914794921875;-0.172458801333352618190275507004116661846637725830078125]
      mask Display: e = 0.06;c1 = [120 150 230]/255;c2 = ([120 150 230]+0)/383;c3 = ([120 150 230]+128)/383;patch([0 1 1 0],[0 0 1 1],c1);patch([0 1 1 1-e 1-e 0+e],[0 0 1 1-e 0+e 0+e],c2);patch([0 0 1 1-e 0+e 0+e],[0 1 1 1-e 1-e 0+e],c3);plot([0 1 1 0 0],[0 0 1 1 0]);disp('Weights');
  "IW{1,1}(6,:)'" : Constant  Value=[0.32104104551125700606206692100386135280132293701171875;2.285731326248320982585937599651515483856201171875;0.387570981917681134376607587910257279872894287109375]
      mask Display: e = 0.06;c1 = [120 150 230]/255;c2 = ([120 150 230]+0)/383;c3 = ([120 150 230]+128)/383;patch([0 1 1 0],[0 0 1 1],c1);patch([0 1 1 1-e 1-e 0+e],[0 0 1 1-e 0+e 0+e],c2);patch([0 0 1 1-e 0+e 0+e],[0 1 1 1-e 1-e 0+e],c3);plot([0 1 1 0 0],[0 0 1 1 0]);disp('Weights');
  "IW{1,1}(7,:)'" : Constant  Value=[-0.2955880691179786357025705001433379948139190673828125;0.7013074604242621745697761070914566516876220703125;-0.4601621601651633142182618030346930027008056640625]
      mask Display: e = 0.06;c1 = [120 150 230]/255;c2 = ([120 150 230]+0)/383;c3 = ([120 150 230]+128)/383;patch([0 1 1 0],[0 0 1 1],c1);patch([0 1 1 1-e 1-e 0+e],[0 0 1 1-e 0+e 0+e],c2);patch([0 0 1 1-e 0+e 0+e],[0 1 1 1-e 1-e 0+e],c3);plot([0 1 1 0 0],[0 0 1 1 0]);disp('Weights');
  "IW{1,1}(8,:)'" : Constant  Value=[0.0159676059342108711547325583524070680141448974609375;0.3310499692983055464168273829272948205471038818359375;-0.5933482783400076954194446443580090999603271484375]
      mask Display: e = 0.06;c1 = [120 150 230]/255;c2 = ([120 150 230]+0)/383;c3 = ([120 150 230]+128)/383;patch([0 1 1 0],[0 0 1 1],c1);patch([0 1 1 1-e 1-e 0+e],[0 0 1 1-e 0+e 0+e],c2);patch([0 0 1 1-e 0+e 0+e],[0 1 1 1-e 1-e 0+e],c3);plot([0 1 1 0 0],[0 0 1 1 0]);disp('Weights');
  "IW{1,1}(9,:)'" : Constant  Value=[0.4014689143571181784153623084421269595623016357421875;-0.93730641180041740501138747276854701340198516845703125;0.29436822918623739564480956687475554645061492919921875]
      mask Display: e = 0.06;c1 = [120 150 230]/255;c2 = ([120 150 230]+0)/383;c3 = ([120 150 230]+128)/383;patch([0 1 1 0],[0 0 1 1],c1);patch([0 1 1 1-e 1-e 0+e],[0 0 1 1-e 0+e 0+e],c2);patch([0 0 1 1-e 0+e 0+e],[0 1 1 1-e 1-e 0+e],c3);plot([0 1 1 0 0],[0 0 1 1 0]);disp('Weights');
  Mux : Mux  Inputs=30
      mask Display: e = 0.06;c1 = [120 150 230]/255;c2 = ([120 150 230]+0)/383;c3 = ([120 150 230]+128)/383;patch([0 1 1 0],[0 0 1 1],c1);patch([0 1 1 1-e 1-e 0+e],[0 0 1 1-e 0+e 0+e],c2);patch([0 0 1 1-e 0+e 0+e],[0 1 1 1-e 1-e 0+e],c3);plot([0 1 1 0 0],[0 0 1 1 0]);disp('Mux');
  dotprod{1..30} (30 alike) : neural/Weight Functions/dotprod
  "iz{1,1}" : Outport
      mask Display: e = 0.06;c1 = [120 230 180]/255;c2 = ([120 230 180]+0)/(256+128);c3 = ([120 230 180]+128)/(256+128);patch([0 1 1 0],[0 0 1 1],c1);patch([0 1 1 1-e 1-e 0+e],[0 0 1 1-e 0+e 0+e],c2);patch([0 0 1 1-e 0+e 0+e],[0 1 1 1-e 1-e 0+e],c3);plot([0 1 1 0 0],[0 0 1 1 0]);
  wires:
  "IW{1,1}(1,:)'"/1 -> dotprod1/1
  "pd{1,1}"/1 -> dotprod1/2, dotprod2/2, dotprod3/2, dotprod4/2, dotprod5/2, dotprod6/2, dotprod7/2, dotprod8/2, dotprod9/2, dotprod10/2, dotprod11/2, dotprod12/2, dotprod13/2, dotprod14/2, dotprod15/2, dotprod16/2, dotprod17/2, dotprod18/2, dotprod19/2, dotprod20/2, dotprod21/2, dotprod22/2, dotprod23/2, dotprod24/2, dotprod25/2, dotprod26/2, dotprod27/2, dotprod28/2, dotprod29/2, dotprod30/2
  dotprod1/1 -> Mux/1
  "IW{1,1}(2,:)'"/1 -> dotprod2/1
  dotprod2/1 -> Mux/2
  "IW{1,1}(3,:)'"/1 -> dotprod3/1
  dotprod3/1 -> Mux/3
  "IW{1,1}(4,:)'"/1 -> dotprod4/1
  dotprod4/1 -> Mux/4
  "IW{1,1}(5,:)'"/1 -> dotprod5/1
  dotprod5/1 -> Mux/5
  "IW{1,1}(6,:)'"/1 -> dotprod6/1
  dotprod6/1 -> Mux/6
  "IW{1,1}(7,:)'"/1 -> dotprod7/1
  dotprod7/1 -> Mux/7
  "IW{1,1}(8,:)'"/1 -> dotprod8/1
  dotprod8/1 -> Mux/8
  "IW{1,1}(9,:)'"/1 -> dotprod9/1
  dotprod9/1 -> Mux/9
  "IW{1,1}(10,:)'"/1 -> dotprod10/1
  dotprod10/1 -> Mux/10
  "IW{1,1}(11,:)'"/1 -> dotprod11/1
  dotprod11/1 -> Mux/11
  "IW{1,1}(12,:)'"/1 -> dotprod12/1
  dotprod12/1 -> Mux/12
  "IW{1,1}(13,:)'"/1 -> dotprod13/1
  dotprod13/1 -> Mux/13
  "IW{1,1}(14,:)'"/1 -> dotprod14/1
  dotprod14/1 -> Mux/14
  "IW{1,1}(15,:)'"/1 -> dotprod15/1
  dotprod15/1 -> Mux/15
  "IW{1,1}(16,:)'"/1 -> dotprod16/1
  dotprod16/1 -> Mux/16
  "IW{1,1}(17,:)'"/1 -> dotprod17/1
  dotprod17/1 -> Mux/17
  "IW{1,1}(18,:)'"/1 -> dotprod18/1
  dotprod18/1 -> Mux/18
  "IW{1,1}(19,:)'"/1 -> dotprod19/1
  dotprod19/1 -> Mux/19
  "IW{1,1}(20,:)'"/1 -> dotprod20/1
  dotprod20/1 -> Mux/20
  "IW{1,1}(21,:)'"/1 -> dotprod21/1
  dotprod21/1 -> Mux/21
  "IW{1,1}(22,:)'"/1 -> dotprod22/1
  dotprod22/1 -> Mux/22
  "IW{1,1}(23,:)'"/1 -> dotprod23/1
  dotprod23/1 -> Mux/23
  "IW{1,1}(24,:)'"/1 -> dotprod24/1
  dotprod24/1 -> Mux/24
  "IW{1,1}(25,:)'"/1 -> dotprod25/1
  dotprod25/1 -> Mux/25
  "IW{1,1}(26,:)'"/1 -> dotprod26/1
  dotprod26/1 -> Mux/26
  "IW{1,1}(27,:)'"/1 -> dotprod27/1
  dotprod27/1 -> Mux/27
  "IW{1,1}(28,:)'"/1 -> dotprod28/1
  dotprod28/1 -> Mux/28
  "IW{1,1}(29,:)'"/1 -> dotprod29/1
  dotprod29/1 -> Mux/29
  "IW{1,1}(30,:)'"/1 -> dotprod30/1
  dotprod30/1 -> Mux/30
  Mux/1 -> "iz{1,1}"/1

== system ACC_FFNN_trainbfg_30_30_30_Nor_Sat_Jan_24_RepFast/Feed-Forward Neural Network/Layer 2/Delays 1 ==
  "p{2}" : Inport  PortDimensions=30
      mask Display: e = 0.06;c1 = [120 230 180]/255;c2 = ([120 230 180]+0)/(256+128);c3 = ([120 230 180]+128)/(256+128);patch([0 1 1 0],[0 0 1 1],c1);patch([0 1 1 1-e 1-e 0+e],[0 0 1 1-e 0+e 0+e],c2);patch([0 0 1 1-e 0+e 0+e],[0 1 1 1-e 1-e 0+e],c3);plot([0 1 1 0 0],[0 0 1 1 0]);
  mux : Mux  Inputs=1
      mask Display: e = 0.06;c1 = [120 150 230]/255;c2 = ([120 150 230]+0)/383;c3 = ([120 150 230]+128)/383;patch([0 1 1 0],[0 0 1 1],c1);patch([0 1 1 1-e 1-e 0+e],[0 0 1 1-e 0+e 0+e],c2);patch([0 0 1 1-e 0+e 0+e],[0 1 1 1-e 1-e 0+e],c3);plot([0 1 1 0 0],[0 0 1 1 0]);disp('Mux')
  "pd{2,1}" : Outport
      mask Display: e = 0.06;c1 = [120 230 180]/255;c2 = ([120 230 180]+0)/(256+128);c3 = ([120 230 180]+128)/(256+128);patch([0 1 1 0],[0 0 1 1],c1);patch([0 1 1 1-e 1-e 0+e],[0 0 1 1-e 0+e 0+e],c2);patch([0 0 1 1-e 0+e 0+e],[0 1 1 1-e 1-e 0+e],c3);plot([0 1 1 0 0],[0 0 1 1 0]);
  wires:
  "p{2}"/1 -> mux/1
  mux/1 -> "pd{2,1}"/1
